simulink model "roll_model_TRUCKSIM_18DOF_REVISED"  (R2023b)
settings: Solver=FixedStepAuto  StartTime=0.0  StopTime=20  FixedStep=0.0005  RelTol=1e-3
StopFcn:
  | save_dataset_18state;
libraries: Solver_SF x1
(part 4 of 5)

== matlab function roll_model_TRUCKSIM_18DOF_REVISED/Subsystem2/MATLAB Function1 ==
  settings: updateMethod=DISCRETE
  data: t input; delta_cmd output; x input; u_prev input; ref12 input; eso_prev input; Mact_cmd output; Fx_req output; omega_ref output; Fz6 output; Fy6 output; eso_next output; dhat5 output; ctrl_diag output; scenario_id input; hitchControlMode input
function [delta_cmd,Mact_cmd,Fx_req,omega_ref,Fz6,Fy6,eso_next,dhat5, ctrl_diag]  = ...
    fcn(t,x,u_prev,ref12,eso_prev,scenario_id,hitchControlMode)
%#codegen
% =========================================================================
% BLOCK 2 - 5-CHANNEL ESO + MODEL-ASSISTED SMC
% DLC11 longitudinal candidate tuned 2026-11-24: reduced peak speed overshoot
%
% Inputs
%   t        scalar [s]
%   x        18x1 TruckSim states
%   u_prev   9x1 previous final actuator command
%   ref12    12x1 output of Block 1
%   eso_prev 10x1 previous ESO state from Unit Delay
%   scenario_id scalar from SAME Constant sent to Block 1 (7 DLC, 8 left, 9 right)
%   hitchControlMode scalar: 0=path + heading only; 1=path + heading + hitch
%   R25 MAT ref12(8) and measured x(5) have SAME gamma sign (rt-rs).
%   Diagnostic-proven; previous forced sign flip is removed for R25.
%
% Outputs
%   delta_cmd  scalar steering [rad]
%   Mact_cmd   scalar active roll moment [N m]
%   Fx_req     scalar requested total longitudinal tire force [N]
%   omega_ref  6x1 wheel-speed reference [rad/s]
%   Fz6        6x1 predicted normal loads [N]
%   Fy6        6x1 predicted lateral tire forces [N]
%   eso_next   10x1 state to feed back through Unit Delay
%   dhat5      5x1 lumped disturbance estimates:
%              [d_vx; d_rt; d_rs; d_roll_t; d_roll_s]
%   ctrl_diag  8x1 [ev eY epsi egamma egamma_dot s_art diag7 LTRf]
%   ctrl_diag(2) = path-normal XY error in scenarios 8/9; global Y error otherwise
%   DLC11 ctrl_diag(7) = unclipped MODEL LTR demand when diagLTRRaw=1/2/3;
%   ctrl_diag(8) remains CLIPPED MODEL front LTR.
%
% Requires:
%   vehicle_18dof_full_roll_road.m
% =========================================================================

Ts=0.01;
% Explicit scalar preallocation helps Simulink Coder resolve output sizes.
delta_cmd=0.0;
Mact_cmd=0.0;
Fx_req=0.0;
omega_ref=zeros(6,1);
Fz6=zeros(6,1);
Fy6=zeros(6,1);
eso_next=zeros(10,1);
dhat5=zeros(5,1);
ctrl_diag=zeros(8,1);

% ===== SINGLE SWITCH FOR ALL SCENARIOS (including DLC11 and JTURN12) =====
rollTestMode = 2.0;   % 0=OFF, 1=rate damping, 2=PD balanced, 3=PD stronger
% Diagnostic ONLY: severe DLC11, select ctrl_diag(7) content:
% 0 = sRoll (old output), 1 = unclipped MODEL front LTR demand,
% 2 = unclipped MODEL rear LTR demand, 3 = unclipped MODEL trailer LTR demand.
% None of these model estimates are TruckSim measured wheel-load LTR.
diagLTRRaw = 1.0;
% Verified test sign: positive IMP_MX_EXT increases positive roll.
% Therefore damping command uses negative feedback of measured roll.
% This actuator currently acts on tractor; trailer LTR must be checked.


%% ========================================================================
% SCENARIO 12 - IDENTICAL OPEN-LOOP STEERING, Mact ON/OFF TEST
% ========================================================================
% This branch deliberately BYPASSES SMC path steering and the ESO/speed
% controller in scenarios 1..11. The same steering is sent in Mode 0/2.
% In TruckSim use internal constant-speed control (40 km/h), and disable
% imported drive torque, so Fx_req=0 doesn't create speed-controller fights.
% CAUTION: yPred(6/7/47) are MODEL LTRs, NOT TruckSim measured wheel loads.
if scenario_id >= 11.5 && scenario_id < 12.5
    % Uses the SINGLE rollTestMode switch at the top of this function.

    vRef = ref12(1);
    muTest = max(ref12(12),0.15);
    % In scenario 12, Block 1 passes steering amplitude in ref12(11).
    % Block 2 has no speed_case input port; no additional wiring needed.
    deltaAmp = min(max(abs(ref12(11)),0.0),8.0*pi/180.0);

    % Right-hand J-turn: smooth 0->-delta, hold, smooth return to zero.
    % 0-4 s straight; 4-6 s ramp; 6-11 s hold; 11-13 s release.
    rise = smoothstep01((t-4.0)/2.0);
    fall = 1.0-smoothstep01((t-11.0)/2.0);
    deltaTarget = -deltaAmp*rise*fall;
    delta_cmd = rate_limit(deltaTarget,u_prev(1),10.0*pi/180.0*Ts);
    delta_cmd = clamp(delta_cmd,-9.0*pi/180.0,9.0*pi/180.0);

    % J-turn is NOT a speed tracking experiment. Block 3 commands no
    % traction/brake. The TruckSim speed driver must use a CONSTANT target.
    Fx_req = 0.0;
    omega_ref(:) = max(x(1),0.0)/0.51;
    eso_next = eso_prev;    % no ESO state update in open-loop branch
    dhat5(:) = 0.0;

    % Use old state vector convention; 18DOF predictor used only to
    % compute physical wheel normal loads and local LTR sensitivity.
    xRoll = x;
    xRoll(5) = x(5);  % gamma=psi_tractor-psi_trailer as model expects
    uZero=u_prev;
    uZero(1)=delta_cmd;
    uZero(2)=0.0;
    uZero(3)=0.0;
    uZero(4:9)=0.0;
    [~,yZero,~,~,~,~,~] = vehicle_18dof_full_roll_road(xRoll,uZero,muTest);

    % Model loads for diagnostic / optional scheduling only.
    % Load transfer computed from this old model may not match the loaded
    % TruckSim configuration. Controller direction is based on measured roll.
    LTRf = yZero(6);
    LTRr = yZero(7);
    LTRmetric = max(abs(LTRf),abs(LTRr));

    [Mact_cmd,rollActivation,sRoll] = active_roll_pd( ...
        x(15),x(16),u_prev(3),LTRmetric,rollTestMode,Ts);

    uPred=uZero;
    uPred(3)=Mact_cmd;
    [~,yPred,~,~,~,~,~]=vehicle_18dof_full_roll_road(xRoll,uPred,muTest);
    for i=1:6
        Fz6(i)=max(yPred(11+i),1.0);
        Fy6(i)=yPred(23+i);
    end
    ctrl_diag(1)=x(1)-vRef;            % actual speed minus 40 km/h
    ctrl_diag(2)=0.0;                 % no lateral-tracking error in J-turn
    ctrl_diag(3)=delta_cmd;           % actual commanded wheel steer [rad]
    ctrl_diag(4)=x(15);               % tractor roll [rad]
    ctrl_diag(5)=x(17);               % trailer roll [rad]
    ctrl_diag(6)=Mact_cmd/12000.0;    % normalized command [-1,1]
    ctrl_diag(7)=yPred(47);           % MODEL trailer LTR
    ctrl_diag(8)=yPred(6);            % MODEL front LTR
    return;
end

% Only scenarios 8/9 receive the quarter-circle tracking modifications.
% Scenarios 1-6 keep their original calculations and gains.
isQuarterTurn = (scenario_id >= 7.5 && scenario_id < 10.5);
isRightLTR = (scenario_id >= 9.5 && scenario_id < 10.5);
isAggDLC = (scenario_id >= 10.5 && scenario_id < 11.5);
isDLCTracking = (scenario_id >= 6.5 && scenario_id < 7.5) || isAggDLC;
% Longitudinal R25 A/B switch: 0 legacy; 1 new bounded-model law.
longitudinalR25Test=1.0;
useBoundedLongitudinal = isDLCTracking || ...
    (isQuarterTurn && longitudinalR25Test>0.5);
% Hitch A/B: set input hitchControlMode = 0 or 1 with a Constant block.
% Only scenarios 8/9 use the A/B mode; scenarios 1-6 retain old hitch logic.
hitchAB = (isQuarterTurn || isAggDLC) && (hitchControlMode >= 0.5);
% R25 measured sign diagnostic (Nov 2026):
% x(5) matches integral(rt-rs) to 8e-6 rad, NOT integral(rs-rt).
% ref12(8) also follows derivative rt_ref-rs_ref.
% Do not negate the MAT gamma or measured x(5) for scenario 8/9.
% Tail-heading priority A/B: 0 = previous path controller, 1 =
% prioritize heading and yaw-rate on the straight section after the turn.
tailHeadingPriorityTest = 1.0;

%% References from Block 1
vx_ref    = ref12(1);
ax_ref    = ref12(2);
Y_ref     = ref12(3);
dY_ref    = ref12(4);
psi_ref   = ref12(5);
rt_ref    = ref12(6);
drt_ref   = ref12(7);
gamma_ref_raw = ref12(8);
% For scenario 8/9, measured x(5) and ref12(8) have the SAME sign.
% Other scenarios retain their original handling (reference unchanged).
gamma_ref_TS = gamma_ref_raw;
rs_ref    = ref12(9);
drs_ref   = ref12(10);
mu_road   = ref12(12);
kappa_ref = ref12(11);

%% States
vx=x(1);
vy=x(2);
rt=x(3);
rs=x(4);
gamma_TS=x(5);             % actual imported hitch signal
if isQuarterTurn || isAggDLC
    % VERIFIED using current TruckSim channels: d(x5)/dt = rt-rs.
    gamma=gamma_TS;        % correct mathematical-model convention
    gamma_ref=gamma_ref_TS; % same sign as MAT ref12(8)
else
    % Preserve pre-existing legacy scenario 1-6 behavior for A/B isolation.
    gamma=-gamma_TS;
    gamma_ref=-gamma_ref_TS;
end
psi=x(6);
Y=x(7);
X=x(8);
phi_t=x(15);
dphi_t=x(16);
phi_s=x(17);
dphi_s=x(18);

%% Vehicle parameters
m_t=5760.0;
m_s=6640.0;
m=m_t+m_s;

Lf=1.305130208;
Lr=2.194869792;
L=Lf+Lr;
Lrs=8.500;

Tf=2.030;
Tr=1.863;
Ts_track=1.863;

Rf=0.51;
Rr=0.51;
Rs=0.51;

%% Current nonlinear model
% The mathematical model uses dgamma = rt-rs (verified in model source).
% For R25 the previous gamma=-x(5) fed an inverted angle into tire/hitch
% geometry and its ESO prediction. Now the R25 model receives x(5).
x_model=x;
x_model(5)=gamma;
[xdot0,y0,~,~,~,~,~]=vehicle_18dof_full_roll_road(x_model,u_prev,mu_road);

%% ========================================================================
% 5-CHANNEL EXTENDED STATE OBSERVER
%
% For each measured channel y:
%   z1_dot = f_model + d_hat + 2*w_o*(y-z1)
%   d_dot  = w_o^2*(y-z1)
%
% This estimates the lumped TruckSim-model mismatch / road disturbance.
% ========================================================================

yMeas=[vx;rt;rs;dphi_t;dphi_s];
fModel=[xdot0(1);xdot0(3);xdot0(4);xdot0(16);xdot0(18)];

wo=[5.0; 0.07; 0.07; 0.07; 0.06];     % Giảm nhẹ wo(1) và wo(2) để bớt dao động cao tần
dLim=[12.0; 5.0; 2.0; 12.0; 12.0];   % Nới rộng dLim(1) và dLim(2) để tránh bị kẹp bão hòa (saturation)

for i=1:5
    iz=2*i-1;
    id=2*i;

    if t<1.5*Ts
        z1=yMeas(i);
        dh=0.0;
    else
        z1=eso_prev(iz);
        dh=eso_prev(id);
    end

    eobs=yMeas(i)-z1;
    beta1=2.0*wo(i);
    beta2=wo(i)*wo(i);

    z1dot=fModel(i)+dh+beta1*eobs;
    dhdot=beta2*eobs;

    z1n=z1+Ts*z1dot;
    dhn=dh+Ts*dhdot;
    dhn=clamp(dhn,-dLim(i),dLim(i));

    eso_next(iz)=z1n;
    eso_next(id)=dhn;
    dhat5(i)=dhn;
end

% Disturbance-corrected model derivatives
% vx=x(1) tracks dxdt(1); y0(34) = dv_x-rt*vy is physical acceleration.
% Use the derivative of the tracked speed in the bounded inversion.
if useBoundedLongitudinal
    ax_model_corr=xdot0(1)+dhat5(1);
else
    ax_model_corr=y0(34)+dhat5(1);
end
dr_model_corr=xdot0(3)+dhat5(2);
drs_model_corr=xdot0(4)+dhat5(3);
ddphi_t_corr=xdot0(16)+dhat5(4);
ddphi_s_corr=xdot0(18)+dhat5(5);

%% ========================================================================
% LONGITUDINAL MA-SMC + ESO
% ========================================================================

ev=vx-vx_ref;

% R25 A/B switch; the remaining controller (ESO/hitch/steering/roll)
% and legacy scenarios are kept unchanged.
% 0: original longitudinal MA-SMC (large model inversion).
% 1: moderate speed feedback + bounded model/ESO correction.

if isAggDLC
    % DLC11 speed-tracking candidate: earlier deceleration, less overshoot.
    % Leave steering/ESO/roll control unchanged.
    kv=2.80;
    Kv=0.20;
    phi_v=0.55;
    ax_pos_cap=min(1.45,0.45*mu_road*9.81);
    ax_neg_cap=min(2.20,0.45*mu_road*9.81);
elseif isDLCTracking
    % Preserve old settings for scenario 7.
    kv=1.80;
    Kv=0.30;
    phi_v=0.50;
    ax_pos_cap=min(1.65,0.45*mu_road*9.81);
    ax_neg_cap=min(1.80,0.45*mu_road*9.81);
elseif useBoundedLongitudinal
    kv=3.50;         % R25 fine-tune: moderate longitudinal feedback
    Kv=0.40;         % m/s^2 robust correction magnitude
    phi_v=0.60;      % m/s boundary layer
    ax_pos_cap=min(3.10,0.45*mu_road*9.81); % exceed reference peak ~2.69 m/s^2
    ax_neg_cap=min(3.00,0.45*mu_road*9.81);
else
    kv=40.0;
    Kv=0.75;
    phi_v=1.4;
    ax_cap=0.60*mu_road*9.81;
    ax_pos_cap=ax_cap;
    ax_neg_cap=ax_cap;
end

ax_des=ax_ref-kv*ev-Kv*satfun(ev/phi_v);
ax_des=clamp(ax_des,-ax_neg_cap,ax_pos_cap);

Fx_prev_total = ...
      u_prev(2)/Rf ...
    - u_prev(4)/Rf-u_prev(5)/Rf ...
    - u_prev(6)/Rr-u_prev(7)/Rr ...
    - u_prev(8)/Rs-u_prev(9)/Rs;

% Original model-based incremental inversion. It can change abruptly when
% tire slip changes, or when drive/brake actuator states change discretely.
Fx_model_raw=Fx_prev_total+m*(ax_des-ax_model_corr);

if useBoundedLongitudinal
    % Nominal tire force with a flat-road drag/rolling-resistance allowance.
    Fx_nominal=m*(ax_des+0.18);

    % Limit the correction from the nonlinear model, ESO and previous torque.
    modelDeltaMax=8000.0;
    if isDLCTracking
        modelDeltaMax=4800.0;
    end
    model_delta=clamp(Fx_model_raw-Fx_nominal,-modelDeltaMax,modelDeltaMax);
    Fx_req=Fx_nominal+0.25*model_delta;
else
    Fx_req=Fx_model_raw;
end

% -------------------------------------------------------------------------
% LONGITUDINAL FORCE REQUEST LIMIT
%
% IMPORTANT:
% The previous +15000 N clamp imposed an unintended drive-torque ceiling:
%   15000*Rf = 15000*0.51 = 7650 Nm
% which is why u9(2) stayed around 7.7-7.8 kNm even though Block 3 allowed
% Tdrive_max = 10000 Nm.
%
% Match the positive force-request ceiling to the physical drive-torque
% ceiling used in Block 3.  Road/tire friction is still limited downstream
% by Block 3, so this does NOT remove the road-aware protection.
% -------------------------------------------------------------------------
Tdrive_req_max = 20000.0;         % [Nm], must match Block 3
Fx_req_pos_max = Tdrive_req_max/Rf; % ~= 39215.69 N
% In the R=25 m turn the entry deceleration can require more than 15 kN.
% Use a bounded road-friction-aware force REQUEST in scenarios 8/9 only.
% This is NOT a guarantee of brake torque: Block 3 still applies tire caps,
% hysteresis, brake filters, rate limits, and its traction/brake interlock.
if isAggDLC
    % Allow realistic controlled deceleration in loaded DLC; final braking
    % is still limited by tire friction in Block 3.
    Fx_req_neg_max = min(26000.0,0.25*mu_road*m*9.81);
elseif isQuarterTurn
    Fx_req_neg_max = min(40000.0,0.50*mu_road*m*9.81);
else
    Fx_req_neg_max = 15000.0; % Original scenarios 1-6 unchanged
end

Fx_req=clamp(Fx_req,-Fx_req_neg_max,Fx_req_pos_max);

% Small force dead zone prevents drive/brake toggling near zero.
if abs(Fx_req)<350.0
    Fx_req=0.0;
end

% ========================================================================
% R25: SMOOTH THE REAL Fx_req SENT TO BLOCK 3 (NOT A DISPLAY-ONLY FILTER)
% ========================================================================
% Fx_req is the LONGITUDINAL force request [N]; Fy6 is lateral tire force.
% 0 = Original Block 2, exact unfiltered Fx_req.
% 1 = Moderate adaptive low-pass + force slew limit.
% 2 = Stronger smoothing for the paper A/B test (experimental).
%
% IMPORTANT: This modifies the actual longitudinal force demand. Keep
% Block 3 unchanged and verify vx and brake/drive performance after tuning.
% Only scenarios 8/9 are modified; scenarios 1-6 remain identical.
forceSmoothMode = 1.0;

% Save the unfiltered request for debugging using a separate To Workspace
% block BEFORE this section if desired. Do NOT mistake alloc_diag(2) for it.
Fx_req_target = Fx_req;

persistent FxReqFilterState FxReqFilterLastT;
if isempty(FxReqFilterState)
    FxReqFilterState = 0.0;
    FxReqFilterLastT = 0.0;
end

% Reset on the beginning of a new simulation, or when time is rewound.
if t <= 1.0e-9 || t < FxReqFilterLastT-1.0e-9
    FxReqFilterState = 0.0;
    FxReqFilterLastT = t;
end

if isQuarterTurn && forceSmoothMode > 0.5
    if t > FxReqFilterLastT+1.0e-9
        dtFx = t-FxReqFilterLastT;
        % A bounded local time step avoids a huge jump if the block skipped
        % a solver step; this block is designed for nominal Ts = 0.01 s.
        dtFx = clamp(dtFx,1.0e-6,0.05);

        if forceSmoothMode < 1.5
            tauFxQuiet  = 0.25;  % [s] nominal  / small speed error
            FxRateQuiet = 24000.0; % [N/s]
        else
            tauFxQuiet  = 0.45;  % [s] stronger smoothing
            FxRateQuiet = 14000.0; % [N/s]
        end

        % During hard acceleration/braking or large speed error, recover
        % quicker authority so the filter does not ruin vx tracking.
        speedTransient = clamp((abs(ev)-0.20)/0.45,0.0,1.0);
        accelTransient = clamp((abs(ax_ref)-0.60)/1.20,0.0,1.0);
        transientWeight = max(speedTransient,accelTransient);
        tauFxFast  = 0.08;     % [s]
        FxRateFast = 60000.0;  % [N/s]
        tauFx  = tauFxQuiet + (tauFxFast-tauFxQuiet)*transientWeight;
        FxRate = FxRateQuiet + (FxRateFast-FxRateQuiet)*transientWeight;

        alphaFx = dtFx/(tauFx+dtFx);
        FxReqCandidate = FxReqFilterState + ...
            alphaFx*(Fx_req_target-FxReqFilterState);
        FxReqFilterState = rate_limit( ...
            FxReqCandidate,FxReqFilterState,FxRate*dtFx);
        FxReqFilterState = clamp( ...
            FxReqFilterState,-Fx_req_neg_max,Fx_req_pos_max);
        FxReqFilterLastT = t;
    end
    Fx_req = FxReqFilterState;
else
    % Mode 0 or non-R25: preserve the original unfiltered command exactly.
    Fx_req = Fx_req_target;
    FxReqFilterState = Fx_req_target;
    FxReqFilterLastT = t;
end

%% ========================================================================
% LATERAL + OPTIMAL-HITCH TRACKING SMC + ESO
% ========================================================================

% QUARTER-TURN: integrate X_ref from the SAME ref12 supplied to Block 2.
% This is essential when using an external MAT reference: its X_ref is NOT
% exactly 20+25*sin(abs(psi_ref)). Incorrect X_ref creates artificial
% cross-track error, especially through a 90-degree turn.
% Guard repeated calls at the same time (minor solver steps); no double count.
persistent XrefInt XrefLastT XrefLastV XrefLastPsi;
if isempty(XrefInt)
    XrefInt=0.0;
    XrefLastT=0.0;
    XrefLastV=vx_ref;
    XrefLastPsi=psi_ref;
end
if t < XrefLastT || t <= 1e-9
    XrefInt=0.0;
    XrefLastT=t;
    XrefLastV=vx_ref;
    XrefLastPsi=psi_ref;
elseif t > XrefLastT
    dtRef=t-XrefLastT;
    % Trapezoidal time integration of the global reference X-velocity.
    XrefInt=XrefInt+0.5*dtRef*( ...
        XrefLastV*cos(XrefLastPsi)+vx_ref*cos(psi_ref));
    XrefLastT=t;
    XrefLastV=vx_ref;
    XrefLastPsi=psi_ref;
end
if isQuarterTurn
    X_ref=XrefInt;

    eX=X-X_ref;
    eYglobal=Y-Y_ref;
    cRef=cos(psi_ref);
    sRef=sin(psi_ref);

    eAlong=cRef*eX+sRef*eYglobal;
    Xdot_actual=vx*cos(psi)-vy*sin(psi);
    Ydot_actual=vx*sin(psi)+vy*cos(psi);
    Xdot_ref=vx_ref*cRef;

    eY=-sRef*eX+cRef*eYglobal;
    eYdot=-sRef*(Xdot_actual-Xdot_ref) ...
          +cRef*(Ydot_actual-dY_ref) ...
          -rt_ref*eAlong;
else
    % Preserve the original lane-change path controller exactly.
    eY=Y-Y_ref;
    eYdot=xdot0(7)-dY_ref;
end

epsi=wrap_pi(psi-psi_ref);
er=rt-rt_ref;

% R25 uses consistent gamma and reference signs in the model and tracker.
egamma=wrap_pi(gamma-gamma_ref);
egamma_TS=wrap_pi(gamma_TS-gamma_ref_TS);

ers=rs-rs_ref;

%% ------------------------------------------------------------------------
% PATH TRACKING SMC
% -------------------------------------------------------------------------
lambda_Y=0.90;
lambda_Ydot=0.82;
lambda_psi=1.00;

s_path = er ...
    +lambda_psi*epsi ...
    +lambda_Y*eY ...
    +lambda_Ydot*eYdot;

Kr      = 2.50;
Kpsi    = 1.20;
KY      = 1.40;
KYdot   = 0.35;
Ksw     = 0.35;
phi_lat = 0.30;

dr_path = drt_ref ...
    -Kr*er ...
    -Kpsi*epsi ...
    -KY*eY ...
    -KYdot*eYdot ...
    -Ksw*satfun(s_path/phi_lat);

%% ------------------------------------------------------------------------
% DEDICATED HITCH / ARTICULATION SMC
%
% Internal-model convention:
%   gamma_dot = r_t-r_s
%
% Therefore:
%   e_gamma_dot=(r_t-r_s)-(r_t_ref-r_s_ref)
%
% This separate surface gives the hitch angle its own damping instead of
% letting it act only as a small correction inside the path surface.
% -------------------------------------------------------------------------
egamma_dot = (rt-rs) - (rt_ref-rs_ref);

%% Second-order damped articulation error dynamics
% Desired behavior:
%   e_gamma_ddot + 2*zeta_art*wn_art*e_gamma_dot
%                 + wn_art^2*e_gamma = 0
%
% zeta_art > 1 gives a slightly overdamped hitch response and is intended
% to reduce the large gamma peaks observed around rapid lane transitions.
wn_art   = 2.00;   % [rad/s]
zeta_art = 1.05;   % slightly overdamped

Kp_art = wn_art*wn_art;
Kd_art = 2.0*zeta_art*wn_art;

% Small robust term: enough for model mismatch, but not large enough to
% dominate the damping law.
eta_art = 0.08;
phi_art = 0.08;

s_art = egamma_dot + wn_art*egamma;

% Desired tractor yaw acceleration required by articulation dynamics.
% drs_model_corr is the nonlinear-model + ESO trailer yaw-acceleration
% estimate.
dr_art = drs_model_corr ...
       +(drt_ref-drs_ref) ...
       -Kd_art*egamma_dot ...
       -Kp_art*egamma ...
       -eta_art*satfun(s_art/phi_art);

% ESO compensation for differential tractor/trailer yaw disturbance.
artic_dist = dhat5(2)-dhat5(3);

%% Limited hitch correction around the path controller
% Do NOT replace the path yaw command with the hitch command.  Instead the
% articulation loop is allowed to add only a bounded correction.
dr_art_corr = dr_art-dr_path;

dr_art_corr_max = 0.35;   % [rad/s^2]
dr_art_corr = clamp( ...
    dr_art_corr,-dr_art_corr_max,dr_art_corr_max);

w_art = 0.50;
% Fair A/B: both R25 modes use the identical path/heading controller.
% Mode 0 removes ALL dedicated hitch action from steering (not just Kdelta_art).
% Mode 1 adds a bounded, secondary hitch correction to the path yaw command.
% The DLC tracking branch uses the path yaw acceleration target.
if isQuarterTurn || isDLCTracking
    if hitchAB
        dr_des=dr_path+w_art*dr_art_corr-0.10*artic_dist;
        s_lat=s_path+0.30*s_art;
    else
        dr_des=dr_path;
        s_lat=s_path;
    end
else
    % Legacy behavior unchanged for scenarios 1-6.
    dr_des=dr_path+w_art*dr_art_corr-0.10*artic_dist;
    s_lat=s_path+0.30*s_art;
end

%% Steering model sensitivity
prev_delta=u_prev(1);
% Speed-dependent steering envelope. High-speed tests retain the conservative
% 5-deg limit; the low-speed figure-eight is allowed larger road-wheel angle.
if isAggDLC
    deltaMax=8.0*pi/180.0;   % severe DLC tracking ceiling
elseif isRightLTR
    deltaMax=14.0*pi/180.0;
elseif isQuarterTurn
    % R=25 m geometric steering is ~7.95 deg. No 12->5 deg step
    % when vx_ref rises through 8 m/s on the exit.
    deltaMax=12.0*pi/180.0;
elseif abs(vx_ref)<8.0
    deltaMax=12.0*pi/180.0;
else
    deltaMax=5.0*pi/180.0;
end
probe=0.20*pi/180.0;

uProbe=u_prev;
deltaProbe=clamp(prev_delta+probe,-deltaMax,deltaMax);
uProbe(1)=deltaProbe;

[xdotProbe,~,~,~,~,~,~]=vehicle_18dof_full_roll_road(x_model,uProbe,mu_road);
dd=deltaProbe-prev_delta;

if abs(dd)>1e-8
    Bdelta=(xdotProbe(3)-xdot0(3))/dd;
else
    Bdelta=0.0;
end

if abs(Bdelta)>0.20
    deltaModel=prev_delta+(dr_des-dr_model_corr)/Bdelta;
else
    deltaModel=prev_delta;
end

deltaModel=clamp(deltaModel,-deltaMax,deltaMax);

% Direct robust steering branch includes only a SMALL hitch damping term.
if isQuarterTurn || isDLCTracking
    % Feedforward from the reference path curvature.
    deltaFF=atan(L*kappa_ref);
else
    deltaFF=atan(L*rt_ref/max(abs(vx),3.0));
end
Kdelta=1.2*pi/180.0;

% Dedicated hitch damping in the direct steering branch.
Kdelta_art = 0.25*pi/180.0;
deltaHitch = 0.0; % secondary hitch term, zero in mode 0

if isAggDLC
    % Severe DLC: two opposite steering events. Moderate hitch support
    % cannot dominate lateral path tracking.
    deltaDirect = deltaFF ...
        -0.31*epsi ...
        -0.16*er ...
        -0.017*eY ...
        -0.045*eYdot ...
        -0.70*pi/180.0*satfun(s_path/0.45);
    if hitchAB
        deltaHitch=clamp(-0.10*egamma-0.05*egamma_dot, ...
                         -0.70*pi/180.0,0.70*pi/180.0);
        deltaDirect=deltaDirect+deltaHitch;
    end
elseif isRightLTR
    % R20 right bend: smooth curvature FF and stronger (bounded) heading/
    % cross-track feedback. No artificial 5deg road-wheel ceiling.
    % Turn is right-hand: negative curvature, heading and steering.
    deltaDirect = deltaFF ...
        -0.34*epsi ...
        -0.15*er ...
        -0.019*eY ...
        -0.038*eYdot ...
        -1.0*pi/180.0*satfun(s_path/0.36);
    if hitchAB
        egClamp=clamp(egamma,-0.40,0.40);
        egDotClamp=clamp(egamma_dot,-0.50,0.50);
        deltaHitch=clamp(-0.18*egClamp-0.08*egDotClamp, ...
                         -1.2*pi/180.0,1.2*pi/180.0);
        deltaDirect=deltaDirect+deltaHitch;
    end
elseif isQuarterTurn
    % Both A/B modes get the same improved yaw/heading response.
    % A modest yaw-rate damping term helps prevent psi overshoot.
    deltaDirect = deltaFF ...
        -0.22*epsi ...
        -0.12*er ...
        -0.010*eY ...
        -0.035*eYdot ...
        -Kdelta*satfun(s_path/phi_lat);

    if hitchAB
        % Secondary articulation controller. With internal gamma=psi_t-psi_s,
        % positive articulation error should REDUCE tractor positive yaw.
        % Positive steering -> positive yaw is assumed, as in deltaFF above.
        egClamp=clamp(egamma,-0.30,0.30);
        egDotClamp=clamp(egamma_dot,-0.50,0.50);
        KgammaP=0.30;     % [rad steering / rad hitch error]
        KgammaD=0.12;     % [s], hitch-rate damping
        deltaHitchRaw=-KgammaP*egClamp-KgammaD*egDotClamp;
        % Heading/path priority: still allow a small hitch correction during
        % large heading error, but never let it dominate the path command.
        headingPriority=clamp(1.0-abs(epsi)/0.35,0.30,1.0);
        deltaHitchMax=2.0*pi/180.0;
        deltaHitch=clamp(headingPriority*deltaHitchRaw, ...
                         -deltaHitchMax,deltaHitchMax);
        deltaDirect=deltaDirect+deltaHitch;
    end
elseif isDLCTracking
    % Each feedback term damps its measured-minus-reference error.
    % Keep articulation out of steering in this path-tracking test.
    deltaDirect = deltaFF ...
        -0.26*epsi ...
        -0.16*er ...
        -0.019*eY ...
        -0.030*eYdot ...
        -Kdelta*satfun(s_path/phi_lat);
else
    % EXACT legacy steering for scenarios 1-6, including old hitch term.
    deltaDirect = deltaFF ...
        -0.18*epsi ...
        -0.01*eY ...
        -0.045*eYdot ...
        -Kdelta*satfun(s_path/phi_lat) ...
        -Kdelta_art*satfun(s_art/phi_art);
end

% -------------------------------------------------------------------------
% R25 EXIT STRAIGHT: HEADING PRIORITY (A/B)
% The recorded problem after 21 s was psi actual > psi_ref and rt > 0,
% while final steering stayed POSITIVE 4-9 deg. At 90 deg the global-X
% cross-track loop can overwhelm heading feedback if X error accumulates.
% Restrict the path correction to +/-1 deg once reference curvature and
% yaw rate are essentially zero. Do not override the steering sign blindly:
% retain signed heading + yaw-rate feedback, and keep small path authority.
% Identical heading law in hitchControlMode 0/1; only hitch term differs.
% -------------------------------------------------------------------------
onExitStraight = false;
if isQuarterTurn && tailHeadingPriorityTest > 0.5
    onExitStraight = abs(psi_ref) > 1.48 && ...
                     abs(kappa_ref) < 0.008 && abs(rt_ref) < 0.025;
    if onExitStraight
        KpsiTail = 0.6;  % steering rad / heading error rad
        KrTail   = 0.4;  % steering rad / yaw-rate error (rad/s)
        dHeading = -KpsiTail*epsi - KrTail*er;
        dPath = clamp(-0.004*eY-0.012*eYdot, ...
                      -1.0*pi/180.0, 1.0*pi/180.0);
        deltaDirect = deltaFF + dHeading + dPath;
        if hitchAB
            % Hitch has LOWER priority than heading after the turn.
            dHitchTail=clamp(deltaHitch, ...
                          -0.70*pi/180.0,0.70*pi/180.0);
            if abs(epsi) > 0.05 && dHitchTail*dHeading < 0.0
                % Suppress a hitch demand opposing correction of a large
                % heading error, rather than turning further from 90 deg.
                dHitchTail=0.0;
            end
            deltaDirect=deltaDirect+dHitchTail;
        end
    end
end

%% MODEL-ASSISTED YAW CORRECTION
% SMC remains the primary tracking controller.
% The nonlinear model and ESO provide a bounded correction.

Breg = 3.0;                   % Regularization [s^-2]
etaModel = 0.20;              % Initial test value
deltaCorrMax = 0.15*pi/180;  % Max correction: 0.15 deg

deltaCorrection = 0.0;

if abs(Bdelta) > 1.0 && ...
   abs(deltaDirect-prev_delta) < 1.0*pi/180

    % Predicted yaw acceleration at direct steering
    drPred = dr_model_corr ...
           + Bdelta*(deltaDirect-prev_delta);

    % Dynamic yaw-acceleration tracking residual.
    % IMPORTANT: use dr_des, not bare drt_ref.  dr_des already contains the
    % bounded hitch/articulation correction; using drt_ref here would bypass
    % most of the dedicated hitch controller.
    eDr = dr_des-drPred;

    % Regularized local model inversion
    deltaCorrection = ...
        (Bdelta/(Bdelta*Bdelta+Breg*Breg))*eDr;

    deltaCorrection = clamp( ...
        deltaCorrection,-deltaCorrMax,deltaCorrMax);
end

% Model-assisted SMC steering
deltaTarget = deltaDirect ...
            + etaModel*deltaCorrection;

deltaTarget = clamp(deltaTarget,-deltaMax,deltaMax);


% Low-mu road: slightly slower steering command slew.
roadScale=clamp(mu_road/0.85,0.35,1.0);
if isAggDLC
    deltaRateMax=16.0*pi/180.0;
elseif isQuarterTurn
    % Keep slew envelope continuous across the reference 8 m/s crossing.
    deltaRateMax=(10.0+5.0*roadScale)*pi/180.0;
elseif isDLCTracking
    % Extra slew headroom for combined DLC feedforward and feedback.
    deltaRateMax=(6.0+4.0*roadScale)*pi/180.0;
elseif abs(vx_ref)<8.0
    deltaRateMax=(10.0+5.0*roadScale)*pi/180.0;
else
    deltaRateMax=(4.5+1.5*roadScale)*pi/180.0;
end

delta_cmd=rate_limit(deltaTarget,prev_delta,deltaRateMax*Ts);
delta_cmd=clamp(delta_cmd,-deltaMax,deltaMax);

%% ========================================================================
% ACTIVE ROLL CONTROL (PD on measured tractor roll + rate)
% ========================================================================
% WHY: A finite-difference dLTR/dM computed after +/-1 clipping returns
% zero at wheel-lift limits, disabling the old actuator at the worst time.
% A/B tests: mode 0 -> Mact_cmd=0; mode 2 -> feedback active.
% No change to steering, ESO, speed control, or Block 3 I/O.
% The sign was identified by +10000/-10000 Nm tests in TruckSim:
% +M shifts measured roll to the positive side.

% TruckSim and 18DOF use matching tractor roll convention only if the
% imported x(15) is the real tractor Roll [rad]. Confirm on a Scope.
uZero=u_prev;
uZero(1)=delta_cmd;
uZero(3)=0.0;
[~,yZero,~,~,~,~,~]=vehicle_18dof_full_roll_road(x_model,uZero,mu_road);
LTRf0=yZero(6);
LTRr0=yZero(7);
LTRs0=yZero(47); %#ok<NASGU>
LTRcurrent=max(abs(LTRf0),abs(LTRr0));

[Mact_cmd,rollActivation,sRoll]=active_roll_pd( ...
    phi_t,dphi_t,u_prev(3),LTRcurrent,rollTestMode,Ts);

% Note: LTRcurrent is just a MODEL estimate; it may saturate at +/-1 and
% does not prove the loaded TruckSim tires have lifted off the road.
% Active feedback is fundamentally on measured phi_t,dphi_t, not LTR slope.
LTRpred=LTRcurrent; %#ok<NASGU>

%% ========================================================================
% MODEL PREDICTION AFTER PRIMARY STEERING + ROLL COMMANDS
% ========================================================================

uPred=u_prev;
uPred(1)=delta_cmd;
uPred(3)=Mact_cmd;
[~,yPred,~,~,~,~,~]=vehicle_18dof_full_roll_road(x_model,uPred,mu_road);

for i=1:6
    Fz6(i)=max(yPred(11+i),1.0);
    Fy6(i)=yPred(23+i);
end

%% ========================================================================
% WHEEL SPEED REFERENCES USING OPTIMAL HITCH REFERENCE
% ========================================================================

VfLx=vx_ref-rt_ref*Tf/2.0;
VfRx=vx_ref+rt_ref*Tf/2.0;
Vfy=rt_ref*Lf;

VfL=VfLx*cos(delta_cmd)+Vfy*sin(delta_cmd);
VfR=VfRx*cos(delta_cmd)+Vfy*sin(delta_cmd);

VrL=vx_ref-rt_ref*Tr/2.0;
VrR=vx_ref+rt_ref*Tr/2.0;

Vxs=vx_ref*cos(gamma_ref);
VsL=Vxs-rs_ref*Ts_track/2.0;
VsR=Vxs+rs_ref*Ts_track/2.0;

omega_ref(1)=max(VfL,0.0)/Rf;
omega_ref(2)=max(VfR,0.0)/Rf;
omega_ref(3)=max(VrL,0.0)/Rr;
omega_ref(4)=max(VrR,0.0)/Rr;
omega_ref(5)=max(VsL,0.0)/Rs;
omega_ref(6)=max(VsR,0.0)/Rs;

%% Diagnostics
ctrl_diag(1)=ev;
ctrl_diag(2)=eY;
ctrl_diag(3)=epsi;
ctrl_diag(4)=egamma_TS; % actual x(5) minus same-sign ref12(8) for R25
ctrl_diag(5)=egamma_dot; % gamma_dot tracking error, measured rt-rs for R25
ctrl_diag(6)=s_art;
ctrl_diag(7)=sRoll;
% DLC11 optional UNSATURATED MODEL load-transfer demand diagnostic.
% Unlike LTR = (FzL-FzR)/(FzL+FzR) with Fz >= 0 clipping,
% this ratio can exceed +/-1.  It is a DEMAND/SEVERITY indicator only;
% it is NOT a physical wheel load ratio once wheel lift starts.
% For actual TruckSim LTR, use TruckSim per-wheel normal forces.
if isAggDLC && diagLTRRaw > 0.5
    Kf_diag = 586026.625861;
    Kr_diag = 435943.669270;
    Ks_diag = 521887.338539;
    Cf_diag = 9075.0;
    Cr_diag = 15000.0;
    Cs_diag = 15000.0;
    etaF_diag = Kf_diag/(Kf_diag+Kr_diag);
    etaR_diag = 1.0-etaF_diag;
    if diagLTRRaw < 1.5
        FzAx_diag = max(yPred(12)+yPred(13),100.0);
        momentRoad = Kf_diag*phi_t+Cf_diag*dphi_t-etaF_diag*Mact_cmd;
        ctrl_diag(7) = 2.0*momentRoad/(2.030*FzAx_diag);
    elseif diagLTRRaw < 2.5
        FzAx_diag = max(yPred(14)+yPred(15),100.0);
        momentRoad = Kr_diag*phi_t+Cr_diag*dphi_t-etaR_diag*Mact_cmd;
        ctrl_diag(7) = 2.0*momentRoad/(1.863*FzAx_diag);
    else
        FzAx_diag = max(yPred(16)+yPred(17),100.0);
        momentRoad = Ks_diag*x(17)+Cs_diag*x(18);
        ctrl_diag(7) = 2.0*momentRoad/(1.863*FzAx_diag);
    end
end
ctrl_diag(8)=yPred(6); % CLIPPED front-axle LTR (MODEL), not TruckSim Fz

% drs_model_corr is intentionally retained as the ESO-corrected trailer
% yaw-acceleration estimate; its disturbance channel enters artic_dist above.

end


function y=satfun(z)
%#codegen
if z>1.0
    y=1.0;
elseif z<-1.0
    y=-1.0;
else
    y=z;
end
end

function y=rate_limit(target,previous,max_step)
%#codegen
d=target-previous;
if d>max_step
    d=max_step;
elseif d<-max_step
    d=-max_step;
end
y=previous+d;
end

function y=clamp(x,lo,hi)
%#codegen
if x>hi
    y=hi;
elseif x<lo
    y=lo;
else
    y=x;
end
end

function a=wrap_pi(a)
%#codegen
a=atan2(sin(a),cos(a));
end

% =========================================================================
% Quintic C2 smoothstep for J-turn actuator reference, MATLAB Coder safe.
% =========================================================================
function h=smoothstep01(z)
%#codegen
z=min(max(z,0.0),1.0);
h=10.0*z*z*z-15.0*z*z*z*z+6.0*z*z*z*z*z;
end

% =========================================================================
% ACTIVE ROLL MOMENT: measured tractor-roll PD with soft gating
% This subfunction is MATLAB Function/Simulink Coder compatible.
% Uses no extra input/output ports and no new Unit Delay blocks.
% =========================================================================
function [Mcmd,activation,sRoll]=active_roll_pd( ...
    phi,phiRate,prevM,LTRmetric,mode,Ts)
%#codegen
% MATLAB Function / Coder-compatible multi-mode comparison controller.
%
% IMPORTANT MODELING LIMITATION:
% A torque that reduces BODY ROLL does not necessarily reduce WHEEL LOAD
% TRANSFER. The 18DOF plant uses Mroad=Kphi*phi+Cphi*dphi-eta*Mact.
% In quasi-static equilibrium, an internal roll moment can be canceled
% by the changed suspension reaction; trailer roll is not directly actuated.
% Therefore do NOT claim a decrease in rollover risk from phi alone.
%
% MODE 0: Mact=0 (reference)
% MODE 1: rate damping only (isolates transient roll oscillation)
% MODE 2: moderate PD (first active roll candidate)
% MODE 3: stronger PD (simulation-only sensitivity test)
%
% Gain units: Kp Nm/rad, Kd Nm*s/rad, torque Nm.
% Sign follows the user's +/-10 kNm test: positive input increases
% positive tractor roll, so negative feedback opposes tractor roll.

sRoll = phi + 0.10*phiRate;
Mcmd = 0.0;
activation = 0.0;
if mode < 0.5
    return;
end

Kp = 0.0;
Kd = 65000.0;
if mode >= 2.5
    Kp = 110000.0;
    Kd = 80000.0;
elseif mode >= 1.5
    Kp = 80000.0;
    Kd = 65000.0;
end

% Keep initial actuator envelope identical for A/B comparisons.
Mmax = 12000.0;
Mrate = 60000.0;
tauM = 0.045;

% Short lead to act before the body roll angle reaches a peak.
% Unlike the original 0.30 s LTR extrapolation, this uses only a
% bounded roll angle/rate and does NOT feed in noisy roll acceleration.
phiLead = phi + 0.075*clamp(phiRate,-0.7,0.7);
phiEff = deadzone_symmetric(phiLead,0.0015);
rateEff = deadzone_symmetric(clamp(phiRate,-0.7,0.7),0.0040);

% DO NOT use the clipped MODEL LTR to control activation.  It is
% unreliable for a loaded TruckSim vehicle with an unchanged 18DOF model.
% LTRmetric remains in the function signature for I/O compatibility.
% LTRmetric intentionally not used as a switching signal.
rollMetric = abs(phiLead)+0.055*abs(rateEff);
activation = smoothstep01((rollMetric-0.0025)/(0.0115-0.0025));

Mraw = -Kp*phiEff-Kd*rateEff;
Mtarget = activation*clamp(Mraw,-Mmax,Mmax);

% Filter and slew directly from last realized command u_prev(3).
% Do not place another filter on Mact in Block 3.
alpha = Ts/(tauM+Ts);
Mfiltered = prevM+alpha*(Mtarget-prevM);
Mcmd = rate_limit(Mfiltered,prevM,Mrate*Ts);
Mcmd = clamp(Mcmd,-Mmax,Mmax);
end

function y=deadzone_symmetric(x,threshold)
%#codegen
if x>threshold
    y=x-threshold;
elseif x<-threshold
    y=x+threshold;
else
    y=0.0;
end
end
